simulink library "Hub_Axis_Lib"  (R2025a)
settings: Solver=ode45  StartTime=0.0  StopTime=10.0  RelTol=1e-3  EnableMultiTasking=on
libraries: fl_lib x4, nesl_utility x3, sm_lib x1
Description:
  | Copyright 2009-2025 The MathWorks, Inc. MathWorks, Inc.
settings Model: Creator=smiller  LastModifiedBy=smiller
settings SolverCC: AlgebraicLoopSolver=TrustRegion
settings DataIOCC: LimitDataPoints=on  SaveFormat=Array  SignalLoggingSaveFormat=ModelDataLogs  ReturnWorkspaceOutputs=off
settings OptimizationCC: ReuseModelBlockBuffer=off  ExpressionDepthLimit=2147483647.0  LifeSpan=inf
settings DebuggingCC: UnderspecifiedInitializationDetection=Classic  MergeDetectMultiDrivingBlocksExec=none  SolverPrmCheckMsg=warning  FcnCallInpInsideContextMsg=warning  UnconnectedInputMsg=warning  UnconnectedOutputMsg=warning  UnconnectedLineMsg=warning  AllowSymbolicDim=off  StateNameClashWarn=warning  PregeneratedLibrarySubsystemCodeDiagnostic=none  SFUnexpectedBacktrackingDiag=warning  SFNoUnconditionalDefaultTransitionDiag=warning  SFExecutionAtInitializationDiag=none  ArithmeticOperatorsInVariantConditions=warning
settings HardwareCC: ProdBitPerPointer=32.0  ProdBitPerSizeT=32.0  ProdBitPerPtrDiffT=32.0  ProdLargestAtomicFloat=None  ProdIntDivRoundTo=Undefined  ProdEndianess=Unspecified  ProdWordSize=32.0  ProdHWDeviceType=32-bit Generic
settings ModelReferenceCC: EnableRefExpFcnMdlSchedulingChecks=on  PropagateSignalLabelsOutOfModel=off
settings SFSimCC: SimUseLocalCustomCode=off  CustomCodeUndefinedFunction=UseInterfaceOnly
settings RTWCC: RTWUseLocalCustomCode=off  GPUComputeCapability=3.5  DLArmComputeVersion=19.05
settings CodeAppCC: StateflowObjectComments=on
settings GRTTargetCC: TargetLangStandard=C89/C90 (ANSI)  CombineOutputUpdateFcns=off  GRTInterface=on
settings ConfigComp: CovMetricSettings=dw  CovSaveCumulativeToWorkspaceVar=on  CovSaveSingleToWorkspaceVar=on  CovExternalEMLEnable=off  CovSFcnEnable=off

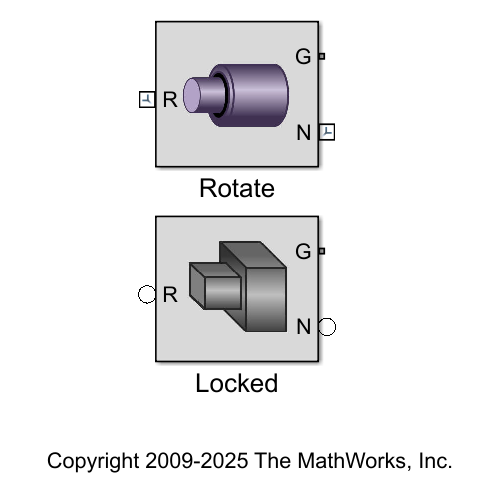
[thumbnail: Simulink's stored preview of the top-level diagram]
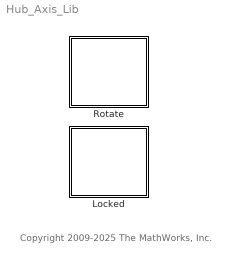
== system Hub_Axis_Lib ==
  note: Copyright 2009-2025 The MathWorks, Inc.
  Locked : Subsystem
      mask Display: image('Hub_Axis_Locked_IMAGE.jpg');
  Rotate : Subsystem
      mask Display: image('Hub_Axis_Rotate_IMAGE.jpg');

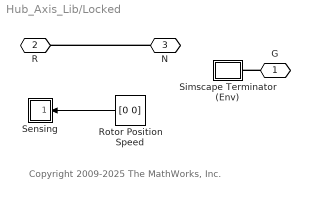
== system Hub_Axis_Lib/Locked ==
  note: Copyright 2009-2025 The MathWorks, Inc.
  Rotor Position Speed : Constant  Value=[0 0]
  Sensing : Subsystem
      mask Display: disp('S');
  Simscape Terminator (Env) : Subsystem
      mask Display:
      | plot([0 0.9],[0.5 0.5]);
      | plot([0.5 0.9],[0.3 0.3]);
      | plot([0.5 0.9],[0.7 0.7]);
      | plot([0.9 0.9],[0.7 0.3]);
  G : PMIOPort  Side=Right
  R : PMIOPort  Port=2  Side=Left
  N : PMIOPort  Port=3  Side=Right
  wires:
  Rotor Position Speed/1 -> Sensing/1(In1)
  connections:
  G/RConn1 -- Simscape Terminator (Env)/LConn1
  N/RConn1 -- R/RConn1

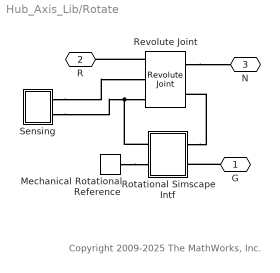
== system Hub_Axis_Lib/Rotate ==
  note: Copyright 2009-2025 The MathWorks, Inc.
  Mechanical Rotational Reference : fl_lib/Mechanical/Rotational Elements/Mechanical Rotational Reference
  Revolute Joint : sm_lib/Joints/Revolute Joint  JointMode=Normal  CompositeWrenchDir=FollowerOnBase  CompositeWrenchFrame=BaseFrame  SenseConstraintForce=off  SenseConstraintTorque=off  SenseTotalForce=off  SenseTotalTorque=off  PositionTargetSpecify=on  PositionTargetPriority=High  PositionTargetValue=0  PositionTargetValueUnits=deg  VelocityTargetSpecify=off  VelocityTargetPriority=High  VelocityTargetValue=0  VelocityTargetValueUnits=deg/s  EquilibriumPosition=0  EquilibriumPositionUnits=deg  SpringStiffness=0  SpringStiffnessUnits=N*m/deg  DampingCoefficient=0  DampingCoefficientUnits=N*m/(deg/s)  LowerLimitSpecify=off  LowerLimitBound=-90  LowerLimitBoundUnits=deg  LowerLimitStiffness=1e4  LowerLimitStiffnessUnits=N*m/deg  LowerLimitDamping=10  LowerLimitDampingUnits=N*m/(deg/s)  LowerLimitTransitionRegionWidth=0.1  LowerLimitTransitionRegionWidthUnits=deg  UpperLimitSpecify=off  UpperLimitBound=90  UpperLimitBoundUnits=deg  UpperLimitStiffness=1e4  UpperLimitStiffnessUnits=N*m/deg  UpperLimitDamping=10  UpperLimitDampingUnits=N*m/(deg/s)  UpperLimitTransitionRegionWidth=0.1  UpperLimitTransitionRegionWidthUnits=deg  TorqueActuationMode=InputTorque  MotionActuationMode=ComputedMotion  SensePosition=on  SenseVelocity=on  SenseAcceleration=off  SenseTorqueForce=off  SenseLowerLimitTorqueForce=off  SenseUpperLimitTorqueForce=off
  Rotational Simscape Intf : Subsystem
  Sensing : Subsystem
  G : PMIOPort  Side=Right
  R : PMIOPort  Port=2  Side=Left
  N : PMIOPort  Port=3  Side=Right
  connections:
  Revolute Joint/RConn1 -- R/RConn1
  Sensing/LConn1 -- Revolute Joint/RConn2
  Revolute Joint/LConn1 -- N/RConn1
  Sensing/LConn2 -- Rotational Simscape Intf/LConn1 -- Revolute Joint/RConn3
  Rotational Simscape Intf/RConn1 -- Revolute Joint/LConn2
  G/RConn1 -- Rotational Simscape Intf/RConn2
  Mechanical Rotational Reference/LConn1 -- Rotational Simscape Intf/LConn2

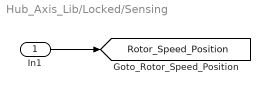
== system Hub_Axis_Lib/Locked/Sensing ==
  In1 : Inport
  tag scope: Rotor_Speed_Position=global
  wires:
  In1/1 -> [Rotor_Speed_Position]

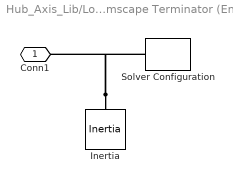
== system Hub_Axis_Lib/Locked/Simscape Terminator (Env) ==
  Inertia : fl_lib/Mechanical/Rotational Elements/Inertia  inertia=1.5e-3 kg*m^2  num_ports=foundation.enum.numPorts2.one  w_specify=on  w_priority=High  w=0 rad/s  w_nominal_specify=off  w_nominal_value=1  w_nominal_unit=rad/s  t_specify=off  t_priority=High  t=0 N*m  t_nominal_specify=off  t_nominal_value=1  t_nominal_unit=N*m
  Solver Configuration : nesl_utility/Solver Configuration  PhysicalDomain=network_engine_domain  SubClassName=solver  LeftPortType=input  RightPortType=generic  Tones=[]  Harmonics=[]  SimulateNoise=off  Profile=off  UseLocalSampling=off  EnableSwitchedLinearOptims=on  FrequencyDomain=off  UseCCode=off  RelTol=0.001  AbsTol=1e-06  MinStep=1e-09  ToWorkspace=off  RevertToSquareIcSolve=off  NumHomotopyIterations=100  PhasorMode=off  PhasorModeNumHarmonics=1  ConsistencySolver=NEWTON_FTOL  IndexReductionMethod=DerivativeReplacement  DoDC=off  ResidualTolerance=1e-9  ConsistencyTolSource=GLOBAL  ConsistencyAbsTol=0.001  ConsistencyRelTol=0.001  ConsistencyTolFactor=0.001  UseLocalSolver=off  LocalSolverChoice=NE_BACKWARD_EULER_ADVANCER  ResolveIndetEquations=on  FunctionEvalNumThread=1  LocalSolverSampleTime=.001  DoFixedCost=off  MaxNonlinIter=3  MaxModeIter=2  ComputeImpulses=off  ImpulseIterations=2  LinearAlgebra=Sparse  LinearAlgebraNumThread=0  EquationFormulation=NE_TIME_EF  DelaysMemoryBudget=1024  AutomaticFiltering=on  FilteringTimeConstant=0.001  PartitionStorageMethod=AS_NEEDED  PartitionMemoryBudget=1024  PartitionMethod=FAST  MultibodyUseLocalSolver=off  MultibodyLocalSolverChoice=ODE1  MultibodyLocalSolverSampleTime=0.001
  Conn1 : PMIOPort  Side=Left
  connections:
  Inertia/LConn1 -- Conn1/RConn1 -- Solver Configuration/RConn1

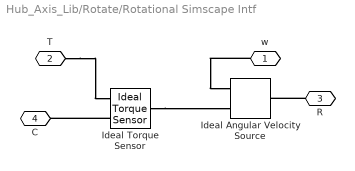
== system Hub_Axis_Lib/Rotate/Rotational Simscape Intf ==
  Ideal Angular Velocity Source : fl_lib/Mechanical/Mechanical Sources/Ideal Angular Velocity Source
  Ideal Torque Sensor : fl_lib/Mechanical/Mechanical Sensors/Ideal Torque Sensor
  w : PMIOPort  Side=Left
  T : PMIOPort  Port=2  Side=Right
  R : PMIOPort  Port=3  Side=Left
  C : PMIOPort  Port=4  Side=Right
  connections:
  Ideal Torque Sensor/RConn1 -- C/RConn1
  R/RConn1 -- Ideal Angular Velocity Source/LConn1
  Ideal Torque Sensor/LConn1 -- Ideal Angular Velocity Source/RConn2
  T/RConn1 -- Ideal Torque Sensor/RConn2
  w/RConn1 -- Ideal Angular Velocity Source/RConn1

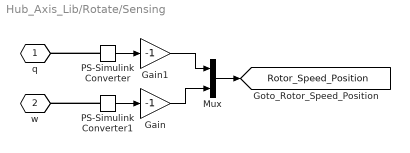
== system Hub_Axis_Lib/Rotate/Sensing ==
  Gain : Gain  Gain=-1
  Gain1 : Gain  Gain=-1
  Mux : Mux  Inputs=2
  PS-Simulink Converter : nesl_utility/PS-Simulink Converter  PhysicalDomain=network_engine_domain  SubClassName=ps_output  LeftPortType=input  RightPortType=output  PseudoPeriodic=off  Frequencies=[]  VectorFormat=1-D array  Unit=deg  AffineConversion=off
  PS-Simulink Converter1 : nesl_utility/PS-Simulink Converter  PhysicalDomain=network_engine_domain  SubClassName=ps_output  LeftPortType=input  RightPortType=output  PseudoPeriodic=off  Frequencies=[]  VectorFormat=1-D array  Unit=rad/s  AffineConversion=off
  q : PMIOPort  Tag=PMCPort  Side=Left
  w : PMIOPort  Tag=PMCPort  Port=2  Side=Left
  tag scope: Rotor_Speed_Position=global
  wires:
  Gain1/1 -> Mux/1
  Gain/1 -> Mux/2
  Mux/1 -> [Rotor_Speed_Position]
  PS-Simulink Converter/1 -> Gain1/1
  PS-Simulink Converter1/1 -> Gain/1
  connections:
  PS-Simulink Converter/LConn1 -- q/RConn1
  PS-Simulink Converter1/LConn1 -- w/RConn1
